simulink model "Module_12S_Test"  (R2025b)
settings: Solver=FixedStepDiscrete  StartTime=0.0  StopTime=360  FixedStep=Ts  RelTol=1e-3
InitFcn:
  | init_BMS
undefined symbols (not defined in the file): Ts
libraries: BMS_Library x1
settings Model: Creator=Khadija  LastModifiedBy=Khadija

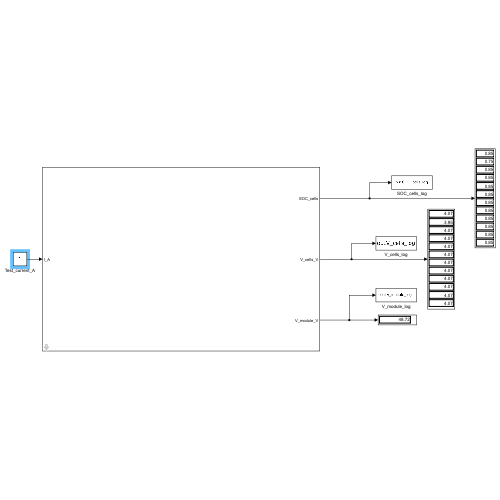
[thumbnail: Simulink's stored preview of the top-level diagram]
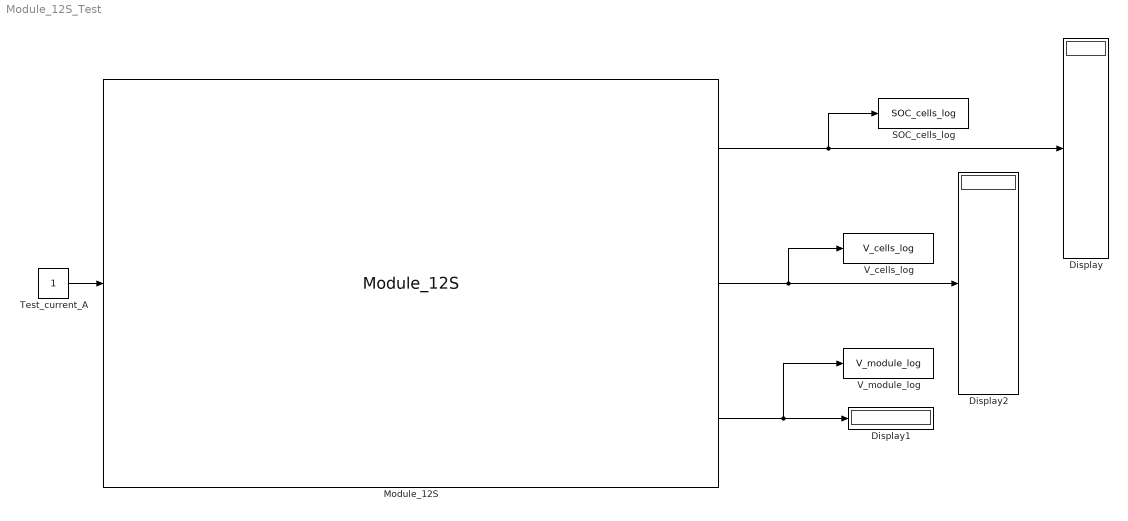
== system Module_12S_Test ==
  Display : Display
  Display1 : Display
  Display2 : Display
  Module_12S : BMS_Library/Module_12S  SOC_init_cells=SOC0_module
  SOC_cells_log : ToWorkspace  VariableName=SOC_cells_log  SaveFormat=Timeseries  SampleTime=-1
  Test_current_A : Constant  SampleTime=Ts
  V_cells_log : ToWorkspace  VariableName=V_cells_log  SaveFormat=Timeseries  SampleTime=-1
  V_module_log : ToWorkspace  VariableName=V_module_log  SaveFormat=Timeseries  SampleTime=-1
  wires:
  Test_current_A/1 -> Module_12S/1
  Module_12S/1 -> SOC_cells_log/1, Display/1
  Module_12S/2 -> V_cells_log/1, Display2/1
  Module_12S/3 -> V_module_log/1, Display1/1
